simulink model "tb_mcu_closed_loop"  (R2026b)
values from neighbouring files (symbols this model uses):
  P = evalin('base', 'P')    [elec_harness.m]    (also in mcu_can1_roundtrip.m; mcu_can2_roundtrip.m; mcu_cl_input.m; mcu_ctrl_harness.m)
  Ts = prm(1)    [mcu_cl_track_dyn.m]    (also in mcu_ctrl_harness.m = evalin('base', tsExpr))
undefined symbols (not defined in the file or in its folder): DiscIntNeverNeededParam
libraries: simulink x57, robotmobilelib x1
(part 2 of 2)

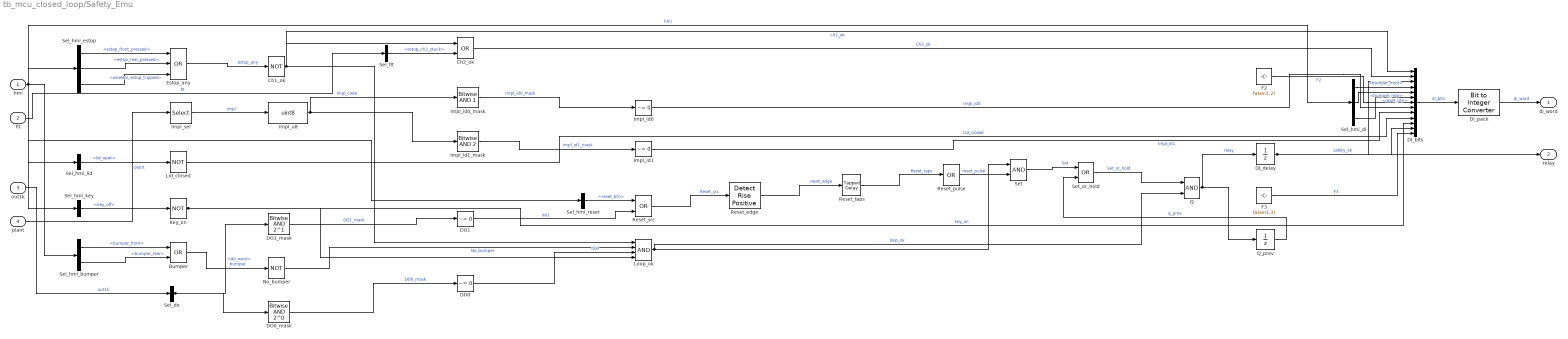
== system tb_mcu_closed_loop/Safety_Emu ==
  hmi : Inport
  flt : Inport  Port=2
  out1k : Inport  Port=3
  plant : Inport  Port=4
  Bumper : Logic  Operator=OR  AllPortsSameDT=off  OutDataTypeStr=boolean
  Ch1_ok : Logic  Operator=NOT  Inputs=1  AllPortsSameDT=off  OutDataTypeStr=boolean
  Ch2_ok : Logic  Operator=OR  AllPortsSameDT=off  OutDataTypeStr=boolean
  DI_delay : UnitDelay  InitialCondition=false  SampleTime=-1
  DO0 : simulink/Logic and Bit Operations/Compare To Zero  relop=~=  OutDataTypeStr=boolean
  DO0_mask : simulink/Logic and Bit Operations/Bitwise Operator  logicop=AND  UseBitMask=on  BitMask=2^0  BitMaskRealWorld=Stored Integer
  DO1 : simulink/Logic and Bit Operations/Compare To Zero  relop=~=  OutDataTypeStr=boolean
  DO1_mask : simulink/Logic and Bit Operations/Bitwise Operator  logicop=AND  UseBitMask=on  BitMask=2^1  BitMaskRealWorld=Stored Integer
  Di_bits : Concatenate  NumInputs=13
  Di_pack : simulink/Logic and Bit Operations/Bit to Integer Converter  nbits=16  bitOrder=LSB first  signedOutputValues=Unsigned  outDtype=uint16  outDtypeSigned=Inherit via internal rule
      settings: LibrarySourceBlock=|
      | commutil2/Bit to Integer
      | Converter
  Estop_any : Logic  Operator=OR  Inputs=3  AllPortsSameDT=off  OutDataTypeStr=boolean
  F2 : Constant  Value=false(1,2)  OutDataTypeStr=boolean  SampleTime=Ts.base
  F3 : Constant  Value=false(1,3)  OutDataTypeStr=boolean  SampleTime=Ts.base
  Impl_id0 : simulink/Logic and Bit Operations/Compare To Zero  relop=~=  OutDataTypeStr=boolean
  Impl_id0_mask : simulink/Logic and Bit Operations/Bitwise Operator  logicop=AND  UseBitMask=on  BitMask=1  BitMaskRealWorld=Stored Integer
  Impl_id1 : simulink/Logic and Bit Operations/Compare To Zero  relop=~=  OutDataTypeStr=boolean
  Impl_id1_mask : simulink/Logic and Bit Operations/Bitwise Operator  logicop=AND  UseBitMask=on  BitMask=2  BitMaskRealWorld=Stored Integer
  Impl_sel : Selector  InputPortWidth=9  IndexOptions=Index vector (dialog)  Indices=7  OutputSizes=1
  Impl_u8 : DataTypeConversion  OutDataTypeStr=uint8  RndMeth=Round
  Key_on : Logic  Operator=NOT  Inputs=1  AllPortsSameDT=off  OutDataTypeStr=boolean
  Lid_closed : Logic  Operator=NOT  Inputs=1  AllPortsSameDT=off  OutDataTypeStr=boolean
  Loop_ok : Logic  Inputs=4  AllPortsSameDT=off  OutDataTypeStr=boolean
  No_bumper : Logic  Operator=NOT  Inputs=1  AllPortsSameDT=off  OutDataTypeStr=boolean
  Q : Logic  AllPortsSameDT=off  OutDataTypeStr=boolean
  Q_prev : UnitDelay  InitialCondition=false  SampleTime=-1
  Reset_edge : simulink/Logic and Bit Operations/Detect Rise Positive  vinit=0  OutDataTypeStr=boolean
  Reset_pulse : Logic  Operator=OR  Inputs=1  AllPortsSameDT=off  OutDataTypeStr=boolean
  Reset_src : Logic  Operator=OR  AllPortsSameDT=off  OutDataTypeStr=boolean
  Reset_taps : simulink/Discrete/Tapped Delay  vinit=0  samptime=-1  NumDelays=round(P.power.safety.t_reset_hold/Ts.base) - 1  DelayOrder=Oldest  includeCurrent=on
  Sel_do : BusSelector  OutputSignals=do_word
  Sel_flt : BusSelector  OutputSignals=estop_ch2_stuck
  Sel_hmi_bumper : BusSelector  OutputSignals=bumper_front,bumper_rear
  Sel_hmi_di : BusSelector  OutputSignals=bumper_front,bumper_rear,reset_btn
  Sel_hmi_estop : BusSelector  OutputSignals=estop_front_pressed,estop_rear_pressed,wireless_estop_tripped
  Sel_hmi_key : BusSelector  OutputSignals=key_off
  Sel_hmi_lid : BusSelector  OutputSignals=lid_open
  Sel_hmi_reset : BusSelector  OutputSignals=reset_btn
  Set : Logic  AllPortsSameDT=off  OutDataTypeStr=boolean
  Set_or_hold : Logic  Operator=OR  AllPortsSameDT=off  OutDataTypeStr=boolean
  di_word : Outport
  relay : Outport  Port=2
  wires:
  hmi/1 -> Sel_hmi_bumper/1, Sel_hmi_key/1, Sel_hmi_reset/1, Sel_hmi_lid/1, Sel_hmi_di/1, Sel_hmi_estop/1  "hmi"
  flt/1 -> Sel_flt/1  "flt"
  out1k/1 -> Sel_do/1  "out1k"
  plant/1 -> Impl_sel/1  "plant"
  Sel_hmi_estop/1 -> Estop_any/1  "<estop_front_pressed>"
  Sel_hmi_estop/2 -> Estop_any/2  "<estop_rear_pressed>"
  Sel_hmi_estop/3 -> Estop_any/3  "<wireless_estop_tripped>"
  Sel_hmi_lid/1 -> Lid_closed/1  "<lid_open>"
  Sel_hmi_key/1 -> Key_on/1  "<key_off>"
  Sel_hmi_bumper/1 -> Bumper/1  "<bumper_front>"
  Sel_hmi_bumper/2 -> Bumper/2  "<bumper_rear>"
  Sel_do/1 -> DO1_mask/1, DO0_mask/1  "<do_word>"
  Estop_any/1 -> Ch1_ok/1  "estop_any"
  Lid_closed/1 -> Di_bits/10  "Lid_closed"
  Key_on/1 -> Di_bits/11, Loop_ok/4  "key_on"
  Bumper/1 -> No_bumper/1  "bumper"
  Impl_sel/1 -> Impl_u8/1  "impl"
  Ch1_ok/1 -> Loop_ok/1, Ch2_ok/1, Di_bits/1  "ch1_ok"
  No_bumper/1 -> Loop_ok/2  "No_bumper"
  DO1_mask/1 -> DO1/1  "DO1_mask"
  DO0_mask/1 -> DO0/1  "DO0_mask"
  Impl_u8/1 -> Impl_id1_mask/1, Impl_id0_mask/1  "impl_code"
  Sel_flt/1 -> Ch2_ok/2  "<estop_ch2_stuck>"
  Ch2_ok/1 -> Di_bits/2  "Ch2_ok"
  DO1/1 -> Reset_src/2  "do1"
  DO0/1 -> Loop_ok/3  "do0"
  Impl_id0_mask/1 -> Impl_id0/1  "Impl_id0_mask"
  Impl_id1_mask/1 -> Impl_id1/1  "Impl_id1_mask"
  Sel_hmi_reset/1 -> Reset_src/1  "<reset_btn>"
  Impl_id0/1 -> Di_bits/8  "Impl_id0"
  Impl_id1/1 -> Di_bits/9  "Impl_id1"
  Reset_src/1 -> Reset_edge/1  "Reset_src"
  Loop_ok/1 -> Set/1, Q/2  "loop_ok"
  Reset_edge/1 -> Reset_taps/1  "reset_edge"
  Reset_taps/1 -> Reset_pulse/1  "Reset_taps"
  Reset_pulse/1 -> Set/2  "reset_pulse"
  Set/1 -> Set_or_hold/1  "Set"
  Set_or_hold/1 -> Q/1  "Set_or_hold"
  Q/1 -> Q_prev/1, DI_delay/1  "relay"
  F2/1 -> Di_bits/7  "F2"
  F3/1 -> Di_bits/13  "F3"
  DI_delay/1 -> Di_bits/3, Di_bits/12, relay/1  "safety_ok"
  Q_prev/1 -> Set_or_hold/2  "q_prev"
  Sel_hmi_di/1 -> Di_bits/4  "<bumper_front>"
  Sel_hmi_di/2 -> Di_bits/5  "<bumper_rear>"
  Sel_hmi_di/3 -> Di_bits/6  "<reset_btn>"
  Di_bits/1 -> Di_pack/1  "di_bits"
  Di_pack/1 -> di_word/1  "di_word"

== matlab function tb_mcu_closed_loop/Plant/Track_dyn ==
  data: v_cmd input; v output; en input; tlim input; pl input; prm input
function v = fcn(v_cmd, en, tlim, pl, prm)
%#codegen
% physical track speeds of the bench (tests/electronics/mcu_cl_track_dyn.m)
v = mcu_cl_track_dyn(v_cmd, en, tlim, pl, prm);
